simulink model "mpc_psm"  (R2026b)
settings: Solver=ode23tb  StopTime=param.sim.simlength  FixedStep=param.glb_time.tc  MaxStep=param.glb_time.tc
values from neighbouring files (symbols this model uses):
  param = struct()    [init_model.m]
undefined symbols (not defined in the file or in its folder): tc
libraries: fl_lib x28, nesl_utility x13, cstblocks_lti x6, lithium_ion_battery x1, dclink_with_center_tap x1, ideal_bridges_lib x1, dead_time_generator_cmos_simulink x1, single_phase_pwm_modulator x1, threephase_inductor_lib x1, simple_flexible_shaft x1, permanent_magnet_synchronous_machine x1
(part 1 of 3)
settings Model: SimulationMode=accelerator  Creator=dbagn  LastModifiedBy=d.bagnara
settings SolverCC: SolverResetMethod=Robust  ZeroCrossControl=DisableAll
settings DataIOCC: DSMLogging=off  ReturnWorkspaceOutputs=off  SaveOutput=off  SaveTime=off  SignalLogging=off
settings OptimizationCC: ReuseModelBlockBuffer=off
settings SFSimCC: CustomCodeUndefinedFunction=ThrowError  DefaultCustomCodeDeterministicFunctions=All
settings SFSimCC: SimCustomHeaderCode=|
  | #include "rpi.h"
  | #include "mavgflt.h"
  | #include "mavgflt_simulink.h"
  | #include "mavgflts.h"
  | #include "mavgflts_simulink.h"
  | #include "dsmavgflt.h"
  | #include "dsmavgflt_simulink.h"
  | #include "bemf_obsv.h"
  | #include "bemf_obsv_simulink.h"
  | #include "bemf_obsv_load_est.h"
  | #include "bemf_obsv_load_est_simulink.h"
  | #include "dqvector_pi.h"
  | #include "dqvector_pi_simulink.h"
  | #include "sv_pwm_simulink.h"
  | #include "sv_pwm.h"
  | #include "first_harmonic_tracker.h"
  | #include "first_harmonic_tracker_simulink.h"
  | #include "dqpll_thyr.h"
  | #include "dqpll_thyr_simulink.h"
  | #include "dqpll_grid.h"
  | #include "dqpll_grid_simulink.h"
settings SFSimCC: SimUserIncludeDirs=|
  | include
  | src
settings SFSimCC: SimUserSources=|
  | "rpi.c"
  | "mavgflt_simulink.c"
  | "mavgflt.c"
  | "mavgflts_simulink.c"
  | "mavgflts.c"
  | "dsmavgflt_simulink.c"
  | "dsmavgflt.c"
  | "bemf_obsv_simulink.c"
  | "bemf_obsv.c"
  | "bemf_obsv_load_est_simulink.c"
  | "bemf_obsv_load_est.c"
  | "dqvector_pi.c"
  | "dqvector_pi_simulink.c"
  | "sv_pwm_simulink.c"
  | "sv_pwm.c"
  | "first_harmonic_tracker_simulink.c"
  | "first_harmonic_tracker.c"
  | "dqpll_thyr_simulink.c"
  | "dqpll_thyr.c"
  | "dqpll_grid_simulink.c"
  | "dqpll_grid.c"
settings RTWCC: DLArmComputeVersion=19.05
settings SimscapeCC: SimscapeUseEnergyAccounting=off

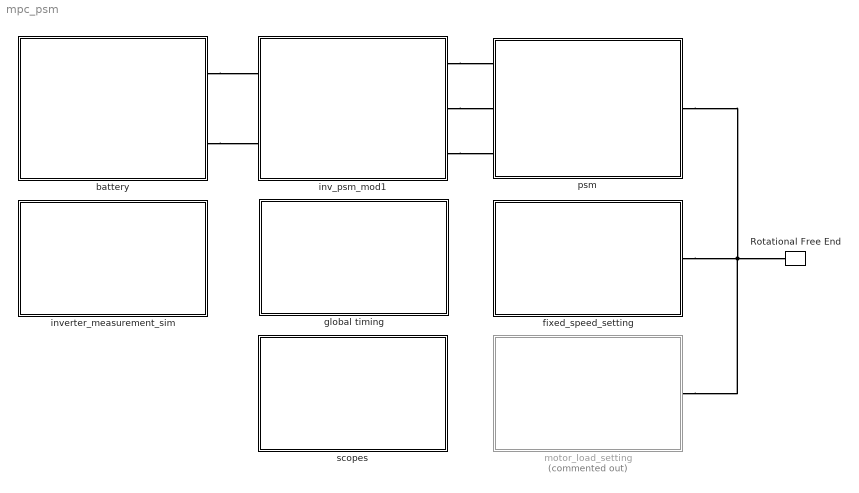
== system mpc_psm ==
  Rotational Free End : fl_lib/Mechanical/Rotational Elements/Rotational Free End  w_specify=off  w_priority=None  w=0 rad/s  w_nominal_specify=off  w_nominal_value=1  w_nominal_unit=rad/s
  battery : Subsystem
  fixed_speed_setting : Subsystem
  global timing : Subsystem
  inv_psm_mod1 : Subsystem
  inverter_measurement_sim : Subsystem
  motor_load_setting : Subsystem  Commented=on
  psm : Subsystem
  scopes : Subsystem
  connections:
  psm/RConn1 -- motor_load_setting/LConn1 -- Rotational Free End/LConn1 -- fixed_speed_setting/LConn1
  inv_psm_mod1/RConn2 -- psm/LConn2
  inv_psm_mod1/RConn1 -- psm/LConn1
  inv_psm_mod1/RConn3 -- psm/LConn3
  battery/RConn1 -- inv_psm_mod1/LConn1
  battery/RConn2 -- inv_psm_mod1/LConn2

== system mpc_psm/battery ==
  Electrical Reference1 : fl_lib/Electrical/Electrical Elements/Electrical Reference
  Solver Configuration : nesl_utility/Solver Configuration  PhysicalDomain=network_engine_domain  SubClassName=solver  LeftPortType=input  RightPortType=generic  Tones=[]  Harmonics=[]  SimulateNoise=off  Profile=off  UseLocalSampling=off  EnableSwitchedLinearOptims=on  FrequencyDomain=off  UseCCode=off  RelTol=0.001  AbsTol=0.001  MinStep=1e-09  ToWorkspace=off  RevertToSquareIcSolve=off  NumHomotopyIterations=100  PhasorMode=off  PhasorModeNumHarmonics=1  ConsistencySolver=NEWTON_FTOL  CanonicalOrdering=UNORDERED  OptimizeIntermediates=UNOPTIMIZED  MulticoreSolverChoice=BACKWARD_EULER  IndexReductionMethod=DerivativeReplacement  DoDC=on  ResidualTolerance=1e-09  ConsistencyTolSource=GLOBAL  ConsistencyAbsTol=0.001  ConsistencyRelTol=0.001  ConsistencyTolFactor=0.001  UseLocalSolver=on  LocalSolverChoice=NE_BACKWARD_EULER_ADVANCER  ResolveIndetEquations=on  FunctionEvalNumThread=1  LocalSolverSampleTime=param.glb_time.tc  DoFixedCost=on  MaxNonlinIter=param.sim.nonlinear_iterations  MaxModeIter=2  ComputeImpulses=off  ImpulseIterations=2  LinearAlgebra=auto  LinearAlgebraNumThread=0  EquationFormulation=NE_TIME_EF  DelaysMemoryBudget=1024  AutomaticFiltering=on  FilteringTimeConstant=0.001  PartitionStorageMethod=AS_NEEDED  PartitionMemoryBudget=1024  PartitionMethod=BALANCED  MultibodyUseLocalSolver=off  MultibodyLocalSolverChoice=ODE1  MultibodyLocalSolverSampleTime=0.001
  To Workspace14 : ToWorkspace  VariableName=battery_data  SampleTime=param.glb_time.tc
      settings: MaxDataPoints=param.glb_time.Nc
  lithium_ion_battery : lithium_ion_battery/lithium_ion_battery  Q=param.battery.pack_1.Q  number_of_cells=param.battery.pack_1.number_of_cells  E_1=param.battery.pack_1.E_1  E0=param.battery.pack_1.E0  E1=param.battery.pack_1.E1  E2=param.battery.pack_1.E2  E3=param.battery.pack_1.E3  Elog=param.battery.pack_1.Elog  R0=param.battery.pack_1.R0  R1=param.battery.pack_1.R1  C1=param.battery.pack_1.C1  M=param.battery.pack_1.M  alpha=param.battery.pack_1.alpha  soc_init=param.battery.pack_1.soc_init  ts_battery=param.glb_time.ts_dab  q1Kalman=param.battery.pack_1.q1Kalman  q2Kalman=param.battery.pack_1.q2Kalman  q3Kalman=param.battery.pack_1.q3Kalman  rKalman=param.battery.pack_1.rKalman  tc=param.glb_time.tc  enable_white_noise_m=0  battery_voltage_init_m=param.battery.nominal_battery_voltage_1
  litium ion battery : Scope
      settings: ActiveDisplayYMinimum=0.16411445056794544  ActiveDisplayYMaximum=0.58434521184828458  DataLoggingVariableName=ScopeData3
  single_phase_ui_measure : Subsystem
  dc+ : PMIOPort  Side=Right
  dc- : PMIOPort  Port=2  Side=Right
  wires:
  lithium_ion_battery/1 -> To Workspace14/1, litium ion battery/1
  connections:
  single_phase_ui_measure/LConn2 -- lithium_ion_battery/RConn2 -- Electrical Reference1/LConn1 -- Solver Configuration/RConn1
  single_phase_ui_measure/RConn1 -- dc+/RConn1
  lithium_ion_battery/RConn1 -- single_phase_ui_measure/LConn1
  dc-/RConn1 -- single_phase_ui_measure/RConn2

== system mpc_psm/fixed_speed_setting ==
  Ideal Angular Velocity Source : fl_lib/Mechanical/Mechanical Sources/Ideal Angular Velocity Source
  Mechanical Rotational Reference : fl_lib/Mechanical/Rotational Elements/Mechanical Rotational Reference
  PS Step1 : fl_lib/Physical Signals/Sources/PS Step  step_time=0.025 s  initial_value=0 rpm  final_value=param.load.rpm_sim rpm
  PS Transfer Function : fl_lib/Physical Signals/Linear Operators/PS Transfer Function  transfer_function_type=foundation.enum.transfer_function_type.lag  T=0.1 s  T1=2 s  T2=1 s  reset_method=foundation.enum.IntegratorResetSpec.None  initial_condition_spec=foundation.enum.IntegratorICSpec.Internal  y0=0 rpm
  shaft : PMIOPort  Side=Left
  connections:
  Mechanical Rotational Reference/LConn1 -- Ideal Angular Velocity Source/RConn2
  PS Step1/RConn1 -- PS Transfer Function/LConn1
  PS Transfer Function/RConn1 -- Ideal Angular Velocity Source/RConn1
  Ideal Angular Velocity Source/LConn1 -- shaft/RConn1

== system mpc_psm/global timing ==
  From9 : From  Commented=on  GotoTag=local_time_corr_afe1
  Unit Delay : UnitDelay  SampleTime=param.glb_time.tc
  Unit Delay1 : UnitDelay  SampleTime=param.glb_time.tc
  time_afe1 : Subsystem  mask{k=param.afe.behav.time_gain_module_1}
      mask prompts: k "Time Gain"
      mask Display:
      | disp('time-gen');
      | port_label('input', 1, 'crt');
      | port_label('output', 1, 'tout');
  time_afe3 : Subsystem  mask{k=1}
      mask prompts: k "Time Gain"
      mask Display:
      | disp('time-gen');
      | port_label('output', 1, 'tout');
  time_inv1 : Subsystem  mask{k=param.inv.behav.time_gain_module_2}
      mask prompts: k "Time Gain"
      mask Display:
      | disp('time-gen');
      | port_label('input', 1, 'crt');
      | port_label('output', 1, 'tout');
  tag scope: time_afe_module_1=global, time_inv_module_1=global, time_master=global
  wires:
  time_afe1/1(Out1) -> [time_afe_module_1]
  time_inv1/1(Out1) -> [time_inv_module_1]
  time_afe3/1(Out1) -> [time_master]
  From9/1 -> Unit Delay/1
  Unit Delay/1 -> time_afe1/1(correction_time)
  [local_time_corr_inv1] -> Unit Delay1/1
  Unit Delay1/1 -> time_inv1/1(correction_time)

== system mpc_psm/inv_psm_mod1 ==
  dclink : Subsystem
  inverter : Subsystem
  inverter_ctrl : Subsystem
  inverter_output_filter : Subsystem
  us_u : PMIOPort  Side=Right
  us_v : PMIOPort  Port=2  Side=Right
  us_w : PMIOPort  Port=3  Side=Right
  udc(+) : PMIOPort  Port=4  Side=Left
  udc(-) : PMIOPort  Port=5  Side=Left
  wires:
  inverter_ctrl/1(cmd_gates) -> inverter/1(cmd_gates)
  connections:
  inverter/LConn2 -- inverter_output_filter/RConn2
  inverter/LConn1 -- inverter_output_filter/RConn1
  inverter/LConn3 -- inverter_output_filter/RConn3
  inverter_output_filter/LConn2 -- us_v/RConn1
  inverter_output_filter/LConn3 -- us_w/RConn1
  inverter_output_filter/LConn1 -- us_u/RConn1
  dclink/RConn1 -- inverter/RConn1
  inverter/RConn2 -- dclink/RConn2
  udc(+)/RConn1 -- dclink/LConn1
  udc(-)/RConn1 -- dclink/LConn2

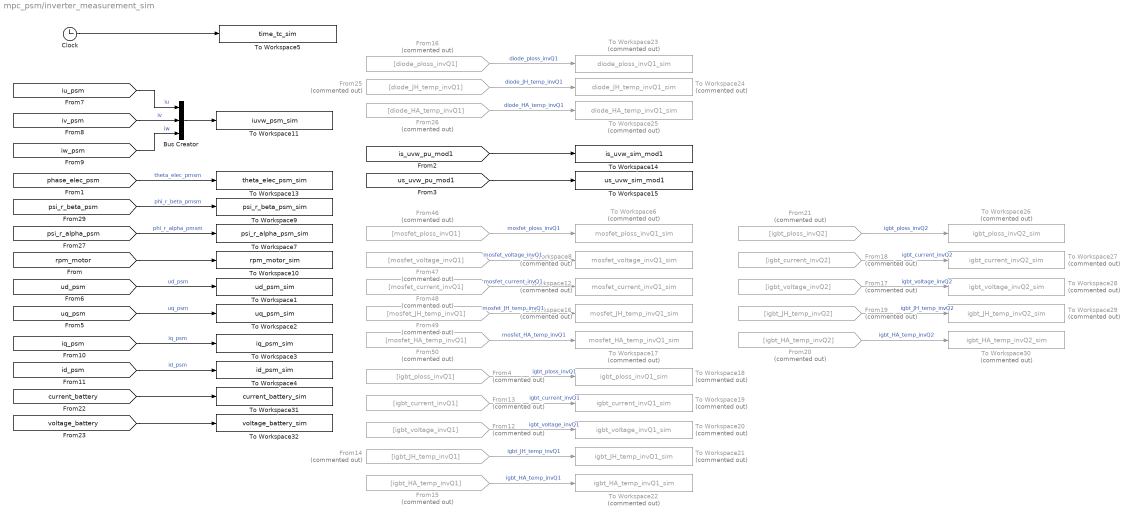
== system mpc_psm/inverter_measurement_sim ==
  Bus Creator : BusCreator  Inputs=3
  Clock : Clock
  From12 : From  Commented=on  GotoTag=igbt_voltage_invQ1
  From13 : From  Commented=on  GotoTag=igbt_current_invQ1
  From14 : From  Commented=on  GotoTag=igbt_JH_temp_invQ1
  From15 : From  Commented=on  GotoTag=igbt_HA_temp_invQ1
  From16 : From  Commented=on  GotoTag=diode_ploss_invQ1
  From17 : From  Commented=on  GotoTag=igbt_voltage_invQ2
  From18 : From  Commented=on  GotoTag=igbt_current_invQ2
  From19 : From  Commented=on  GotoTag=igbt_JH_temp_invQ2
  From20 : From  Commented=on  GotoTag=igbt_HA_temp_invQ2
  From21 : From  Commented=on  GotoTag=igbt_ploss_invQ2
  From25 : From  Commented=on  GotoTag=diode_JH_temp_invQ1
  From26 : From  Commented=on  GotoTag=diode_HA_temp_invQ1
  From4 : From  Commented=on  GotoTag=igbt_ploss_invQ1
  From46 : From  Commented=on  GotoTag=mosfet_ploss_invQ1
  From47 : From  Commented=on  GotoTag=mosfet_voltage_invQ1
  From48 : From  Commented=on  GotoTag=mosfet_current_invQ1
  From49 : From  Commented=on  GotoTag=mosfet_JH_temp_invQ1
  From50 : From  Commented=on  GotoTag=mosfet_HA_temp_invQ1
  To Workspace1 : ToWorkspace  VariableName=ud_psm_sim  SampleTime=param.glb_time.tc
      settings: MaxDataPoints=param.glb_time.Nc  Save2DSignal=2-D array (concatenate along first dimension)
  To Workspace10 : ToWorkspace  VariableName=rpm_motor_sim  SampleTime=param.glb_time.tc
      settings: MaxDataPoints=param.glb_time.Nc  Save2DSignal=2-D array (concatenate along first dimension)
  To Workspace11 : ToWorkspace  VariableName=iuvw_psm_sim  SampleTime=param.glb_time.tc
      settings: MaxDataPoints=param.glb_time.Nc  Save2DSignal=2-D array (concatenate along first dimension)
  To Workspace12 : ToWorkspace  Commented=on  VariableName=mosfet_current_invQ1_sim  SampleTime=tc
      settings: MaxDataPoints=Nc  Save2DSignal=2-D array (concatenate along first dimension)
  To Workspace13 : ToWorkspace  VariableName=theta_elec_psm_sim  SampleTime=param.glb_time.tc
      settings: MaxDataPoints=param.glb_time.Nc  Save2DSignal=2-D array (concatenate along first dimension)
  To Workspace14 : ToWorkspace  VariableName=is_uvw_sim_mod1  SampleTime=param.glb_time.tc
      settings: MaxDataPoints=param.glb_time.Nc  Save2DSignal=2-D array (concatenate along first dimension)
  To Workspace15 : ToWorkspace  VariableName=us_uvw_sim_mod1  SampleTime=param.glb_time.tc
      settings: MaxDataPoints=param.glb_time.Nc  Save2DSignal=2-D array (concatenate along first dimension)
  To Workspace16 : ToWorkspace  Commented=on  VariableName=mosfet_JH_temp_invQ1_sim  SampleTime=tc
      settings: MaxDataPoints=Nc  Save2DSignal=2-D array (concatenate along first dimension)
  To Workspace17 : ToWorkspace  Commented=on  VariableName=mosfet_HA_temp_invQ1_sim  SampleTime=tc
      settings: MaxDataPoints=Nc  Save2DSignal=2-D array (concatenate along first dimension)
  To Workspace18 : ToWorkspace  Commented=on  VariableName=igbt_ploss_invQ1_sim  SampleTime=param.glb_time.tc
      settings: MaxDataPoints=param.glb_time.Nc  Save2DSignal=2-D array (concatenate along first dimension)
  To Workspace19 : ToWorkspace  Commented=on  VariableName=igbt_current_invQ1_sim  SampleTime=param.glb_time.tc
      settings: MaxDataPoints=param.glb_time.Nc  Save2DSignal=2-D array (concatenate along first dimension)
  To Workspace2 : ToWorkspace  VariableName=uq_psm_sim  SampleTime=param.glb_time.tc
      settings: MaxDataPoints=param.glb_time.Nc  Save2DSignal=2-D array (concatenate along first dimension)
  To Workspace20 : ToWorkspace  Commented=on  VariableName=igbt_voltage_invQ1_sim  SampleTime=param.glb_time.tc
      settings: MaxDataPoints=param.glb_time.Nc  Save2DSignal=2-D array (concatenate along first dimension)
  To Workspace21 : ToWorkspace  Commented=on  VariableName=igbt_JH_temp_invQ1_sim  SampleTime=param.glb_time.tc
      settings: MaxDataPoints=param.glb_time.Nc  Save2DSignal=2-D array (concatenate along first dimension)
  To Workspace22 : ToWorkspace  Commented=on  VariableName=igbt_HA_temp_invQ1_sim  SampleTime=param.glb_time.tc
      settings: MaxDataPoints=param.glb_time.Nc  Save2DSignal=2-D array (concatenate along first dimension)
  To Workspace23 : ToWorkspace  Commented=on  VariableName=diode_ploss_invQ1_sim  SampleTime=param.glb_time.tc
      settings: MaxDataPoints=param.glb_time.Nc
  To Workspace24 : ToWorkspace  Commented=on  VariableName=diode_JH_temp_invQ1_sim  SampleTime=param.glb_time.tc
      settings: MaxDataPoints=param.glb_time.Nc
  To Workspace25 : ToWorkspace  Commented=on  VariableName=diode_HA_temp_invQ1_sim  SampleTime=param.glb_time.tc
      settings: MaxDataPoints=param.glb_time.Nc
  To Workspace26 : ToWorkspace  Commented=on  VariableName=igbt_ploss_invQ2_sim  SampleTime=param.glb_time.tc
      settings: MaxDataPoints=param.glb_time.Nc  Save2DSignal=2-D array (concatenate along first dimension)
  To Workspace27 : ToWorkspace  Commented=on  VariableName=igbt_current_invQ2_sim  SampleTime=param.glb_time.tc
      settings: MaxDataPoints=param.glb_time.Nc  Save2DSignal=2-D array (concatenate along first dimension)
  To Workspace28 : ToWorkspace  Commented=on  VariableName=igbt_voltage_invQ2_sim  SampleTime=param.glb_time.tc
      settings: MaxDataPoints=param.glb_time.Nc  Save2DSignal=2-D array (concatenate along first dimension)
  To Workspace29 : ToWorkspace  Commented=on  VariableName=igbt_JH_temp_invQ2_sim  SampleTime=param.glb_time.tc
      settings: MaxDataPoints=param.glb_time.Nc  Save2DSignal=2-D array (concatenate along first dimension)
  To Workspace3 : ToWorkspace  VariableName=iq_psm_sim  SampleTime=param.glb_time.tc
      settings: MaxDataPoints=param.glb_time.Nc  Save2DSignal=2-D array (concatenate along first dimension)
  To Workspace30 : ToWorkspace  Commented=on  VariableName=igbt_HA_temp_invQ2_sim  SampleTime=param.glb_time.tc
      settings: MaxDataPoints=param.glb_time.Nc  Save2DSignal=2-D array (concatenate along first dimension)
  To Workspace31 : ToWorkspace  VariableName=current_battery_sim  SampleTime=param.glb_time.tc
      settings: MaxDataPoints=param.glb_time.Nc  Save2DSignal=2-D array (concatenate along first dimension)
  To Workspace32 : ToWorkspace  VariableName=voltage_battery_sim  SampleTime=param.glb_time.tc
      settings: MaxDataPoints=param.glb_time.Nc  Save2DSignal=2-D array (concatenate along first dimension)
  To Workspace4 : ToWorkspace  VariableName=id_psm_sim  SampleTime=param.glb_time.tc
      settings: MaxDataPoints=param.glb_time.Nc  Save2DSignal=2-D array (concatenate along first dimension)
  To Workspace5 : ToWorkspace  VariableName=time_tc_sim  SampleTime=param.glb_time.tc
      settings: MaxDataPoints=param.glb_time.Nc  Save2DSignal=2-D array (concatenate along first dimension)
  To Workspace6 : ToWorkspace  Commented=on  VariableName=mosfet_ploss_invQ1_sim  SampleTime=tc
      settings: MaxDataPoints=Nc  Save2DSignal=2-D array (concatenate along first dimension)
  To Workspace7 : ToWorkspace  VariableName=psi_r_alpha_psm_sim  SampleTime=param.glb_time.tc
      settings: MaxDataPoints=param.glb_time.Nc  Save2DSignal=2-D array (concatenate along first dimension)
  To Workspace8 : ToWorkspace  Commented=on  VariableName=mosfet_voltage_invQ1_sim  SampleTime=tc
      settings: MaxDataPoints=Nc  Save2DSignal=2-D array (concatenate along first dimension)
  To Workspace9 : ToWorkspace  VariableName=psi_r_beta_psm_sim  SampleTime=param.glb_time.tc
      settings: MaxDataPoints=param.glb_time.Nc  Save2DSignal=2-D array (concatenate along first dimension)
  wires:
  [psi_r_alpha_psm] -> To Workspace7/1  "phi_r_alpha_pmsm"
  [psi_r_beta_psm] -> To Workspace9/1  "phi_r_beta_pmsm"
  [rpm_motor] -> To Workspace10/1
  [iv_psm] -> Bus Creator/2  "iv"
  [iw_psm] -> Bus Creator/3  "iw"
  [iu_psm] -> Bus Creator/1  "iu"
  Bus Creator/1 -> To Workspace11/1
  [phase_elec_psm] -> To Workspace13/1  "theta_elec_pmsm"
  [ud_psm] -> To Workspace1/1  "ud_psm"
  [uq_psm] -> To Workspace2/1  "uq_psm"
  [iq_psm] -> To Workspace3/1  "iq_psm"
  [id_psm] -> To Workspace4/1  "id_psm"
  Clock/1 -> To Workspace5/1
  From46/1 -> To Workspace6/1  "mosfet_ploss_invQ1"
  From49/1 -> To Workspace16/1  "mosfet_JH_temp_invQ1"
  From50/1 -> To Workspace17/1  "mosfet_HA_temp_invQ1"
  [is_uvw_pu_mod1] -> To Workspace14/1
  [us_uvw_pu_mod1] -> To Workspace15/1
  From47/1 -> To Workspace8/1  "mosfet_voltage_invQ1"
  From48/1 -> To Workspace12/1  "mosfet_current_invQ1"
  From4/1 -> To Workspace18/1  "igbt_ploss_invQ1"
  From13/1 -> To Workspace19/1  "igbt_current_invQ1"
  From12/1 -> To Workspace20/1  "igbt_voltage_invQ1"
  From14/1 -> To Workspace21/1  "igbt_JH_temp_invQ1"
  From15/1 -> To Workspace22/1  "igbt_HA_temp_invQ1"
  From16/1 -> To Workspace23/1  "diode_ploss_invQ1"
  From25/1 -> To Workspace24/1  "diode_JH_temp_invQ1"
  From26/1 -> To Workspace25/1  "diode_HA_temp_invQ1"
  From20/1 -> To Workspace30/1  "igbt_HA_temp_invQ2"
  From19/1 -> To Workspace29/1  "igbt_JH_temp_invQ2"
  From17/1 -> To Workspace28/1  "igbt_voltage_invQ2"
  From18/1 -> To Workspace27/1  "igbt_current_invQ2"
  From21/1 -> To Workspace26/1  "igbt_ploss_invQ2"
  [current_battery] -> To Workspace31/1
  [voltage_battery] -> To Workspace32/1

== system mpc_psm/motor_load_setting ==
  Ideal Torque Source : fl_lib/Mechanical/Mechanical Sources/Ideal Torque Source
  Inertia : fl_lib/Mechanical/Rotational Elements/Inertia  inertia=param.load.external_load_inertia kg*m^2  num_ports=foundation.enum.numPorts2.one  w_specify=off  w_priority=High  w=0 rad/s  w_nominal_specify=off  w_nominal_value=1  w_nominal_unit=rad/s  t_specify=off  t_priority=None  t=0 N*m  t_nominal_specify=off  t_nominal_value=1  t_nominal_unit=N*m
  Mechanical Rotational Reference : fl_lib/Mechanical/Rotational Elements/Mechanical Rotational Reference
  PS Step : fl_lib/Physical Signals/Sources/PS Step  step_time=param.sim.load_step_time s  initial_value=1 N*m  final_value=1 N*m
  PS Transfer Function : fl_lib/Physical Signals/Linear Operators/PS Transfer Function  transfer_function_type=foundation.enum.transfer_function_type.lag  T=1 s  T1=2 s  T2=1 s  reset_method=foundation.enum.IntegratorResetSpec.None  initial_condition_spec=foundation.enum.IntegratorICSpec.Internal  y0=0 N*m
  flexible_shaft : simple_flexible_shaft/flexible_shaft  b1=1  b2=1  J1=1  J2=1  b_displacement=1  k_displacement=1e5
  shaft : PMIOPort  Side=Left
  connections:
  Ideal Torque Source/LConn1 -- flexible_shaft/RConn1 -- Inertia/LConn1
  Ideal Torque Source/RConn2 -- Mechanical Rotational Reference/LConn1
  PS Transfer Function/RConn1 -- Ideal Torque Source/RConn1
  PS Step/RConn1 -- PS Transfer Function/LConn1
  flexible_shaft/LConn1 -- shaft/RConn1

== system mpc_psm/psm ==
  Bus Selector1 : BusSelector  OutputSignals=omega_mech (rpm)
  Constant : Constant  Value=param.psm.machine.psi_m
  Simulink-PS Converter3 : nesl_utility/Simulink-PS Converter  PhysicalDomain=network_engine_domain  SubClassName=ps_input  LeftPortType=input  RightPortType=output  PseudoPeriodic=off  Frequencies=[]  NoiseDistribution=none  NoiseParameters=[]  Unit=V*s  AffineConversion=on  FilteringAndDerivatives=provide  SimscapeFilterOrder=1  InputFilterTimeConstant=0.001  UdotUserProvided=0
  synchronous_motor : Subsystem
  u : PMIOPort  Side=Left
  v : PMIOPort  Port=2  Side=Left
  w : PMIOPort  Port=3  Side=Left
  shaft : PMIOPort  Port=4  Side=Right
  tag scope: rpm_motor=global
  wires:
  synchronous_motor/1(motor_data) -> Bus Selector1/1
  Bus Selector1/1 -> [rpm_motor]  "<omega_mech (rpm)>"
  Constant/1 -> Simulink-PS Converter3/1
  connections:
  synchronous_motor/LConn1 -- u/RConn1
  Simulink-PS Converter3/RConn1 -- synchronous_motor/LConn4
  synchronous_motor/LConn3 -- w/RConn1
  synchronous_motor/LConn2 -- v/RConn1
  shaft/RConn1 -- synchronous_motor/RConn1

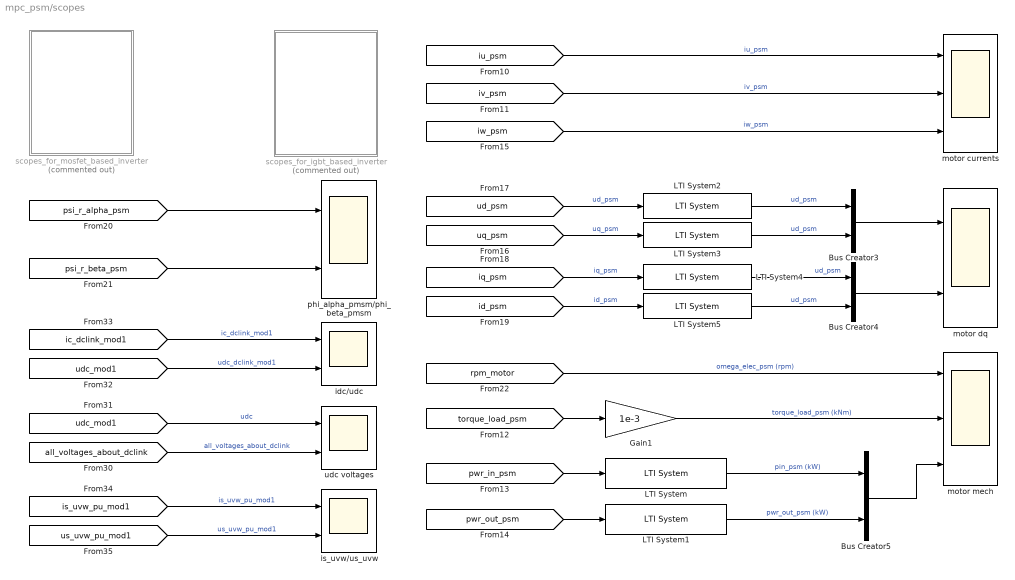
== system mpc_psm/scopes ==
  Bus Creator3 : BusCreator  Inputs=2
  Bus Creator4 : BusCreator  Inputs=2
  Bus Creator5 : BusCreator  Inputs=2
  Gain1 : Gain  Gain=1e-3
  LTI System{,1..5} (6 alike) : cstblocks_lti/LTI System  sys=param.ctrl.filters.inv.SOF_50Hz.ss_c  IC=[]  PadeOrder=0
  idc/udc : Scope  NumInputPorts=2
      settings: SampleTime=param.glb_time.tc  ActiveDisplayYMinimum=-429.79232670429462  ActiveDisplayYMaximum=486.89839586541632  DataLoggingVariableName=ScopeData23
  is_uvw/us_uvw : Scope  NumInputPorts=2
      settings: SampleTime=param.glb_time.tc  ActiveDisplayYMinimum=-4.0901889520524559  ActiveDisplayYMaximum=4.1379165768312332  DataLoggingVariableName=ScopeData25
  motor currents : Scope  NumInputPorts=3
      settings: SampleTime=param.glb_time.tc  ActiveDisplayYMinimum=58.424845691421581  ActiveDisplayYMaximum=93.288598080369269  DataLoggingVariableName=ScopeData17
  motor dq : Scope  NumInputPorts=2
      settings: SampleTime=param.glb_time.tc  ActiveDisplayYMinimum=-581.89506711994022  ActiveDisplayYMaximum=671.86127351087941  DataLoggingVariableName=ScopeData18
  motor mech : Scope  NumInputPorts=3
      settings: SampleTime=param.glb_time.tc  ActiveDisplayYMinimum=17.183598515360881  ActiveDisplayYMaximum=17.193981269957806  DataLoggingVariableName=ScopeData11
  phi_alpha_pmsm/phi_beta_pmsm : Scope  NumInputPorts=2
      settings: SampleTime=param.glb_time.tc  ActiveDisplayYMinimum=-4.800821748013445  ActiveDisplayYMaximum=4.8008423854253959  DataLoggingVariableName=ScopeData19
  scopes_for_igbt_based_inverter : Subsystem  Commented=on
  scopes_for_mosfet_based_inverter : Subsystem  Commented=on
  udc voltages : Scope  NumInputPorts=2
      settings: SampleTime=param.glb_time.tc  ActiveDisplayYMinimum=1171.2930142420437  ActiveDisplayYMaximum=1182.3226675773467  DataLoggingVariableName=ScopeData24
  wires:
  [torque_load_psm] -> Gain1/1
  [pwr_out_psm] -> LTI System1/1
  Bus Creator4/1 -> motor dq/2
  LTI System/1 -> Bus Creator5/1  "pin_psm (kW)"
  LTI System1/1 -> Bus Creator5/2  "pwr_out_psm (kW)"
  [iw_psm] -> motor currents/3  "iw_psm"
  Gain1/1 -> motor mech/2  "torque_load_psm (kNm)"
  [id_psm] -> LTI System5/1  "id_psm"
  [psi_r_alpha_psm] -> phi_alpha_pmsm/phi_beta_pmsm/1
  [iv_psm] -> motor currents/2  "iv_psm"
  Bus Creator3/1 -> motor dq/1
  [uq_psm] -> LTI System3/1  "uq_psm"
  [iu_psm] -> motor currents/1  "iu_psm"
  Bus Creator5/1 -> motor mech/3
  [ud_psm] -> LTI System2/1  "ud_psm"
  [iq_psm] -> LTI System4/1  "iq_psm"
  [rpm_motor] -> motor mech/1  "omega_elec_psm (rpm)"
  [pwr_in_psm] -> LTI System/1
  [psi_r_beta_psm] -> phi_alpha_pmsm/phi_beta_pmsm/2
  [udc_mod1] -> udc voltages/1  "udc"
  [ic_dclink_mod1] -> idc/udc/1  "ic_dclink_mod1"
  [udc_mod1] -> idc/udc/2  "udc_dclink_mod1"
  [all_voltages_about_dclink] -> udc voltages/2  "all_voltages_about_dclink"
  [is_uvw_pu_mod1] -> is_uvw/us_uvw/1  "is_uvw_pu_mod1"
  [us_uvw_pu_mod1] -> is_uvw/us_uvw/2  "us_uvw_pu_mod1"
  LTI System2/1 -> Bus Creator3/1  "ud_psm"
  LTI System3/1 -> Bus Creator3/2  "ud_psm"
  LTI System4/1 -> Bus Creator4/1  "ud_psm"
  LTI System5/1 -> Bus Creator4/2  "ud_psm"

== system mpc_psm/battery/single_phase_ui_measure ==
  Bus Creator : BusCreator  Inputs=2
  Current Sensor : fl_lib/Electrical/Electrical Sensors/Current Sensor
  Selector : Selector  InputPortWidth=2  IndexOptions=Index vector (dialog)  Indices=2  OutputSizes=1  RuntimeRangeChecks=off
  Selector1 : Selector  InputPortWidth=2  IndexOptions=Index vector (dialog)  Indices=1  OutputSizes=1  RuntimeRangeChecks=off
  Voltage Sensor : fl_lib/Electrical/Electrical Sensors/Voltage Sensor
  dab input modA : Scope  NumInputPorts=2
      settings: SampleTime=param.glb_time.tc  ActiveDisplayYMinimum=-0.63173529794617089  ActiveDisplayYMaximum=0.79076436133006256  DataLoggingVariableName=ScopeData2
  iph : nesl_utility/PS-Simulink Converter  PhysicalDomain=network_engine_domain  SubClassName=ps_output  LeftPortType=input  RightPortType=output  PseudoPeriodic=off  Frequencies=[]  VectorFormat=1-D array  Unit=A  AffineConversion=off
  uph : nesl_utility/PS-Simulink Converter  PhysicalDomain=network_engine_domain  SubClassName=ps_output  LeftPortType=input  RightPortType=output  PseudoPeriodic=off  Frequencies=[]  VectorFormat=1-D array  Unit=V  AffineConversion=off
  Udc(+) : PMIOPort  Side=Left
  udc(+) : PMIOPort  Port=2  Side=Right
  Udc(-) : PMIOPort  Port=3  Side=Left
  udc(-) : PMIOPort  Port=4  Side=Right
  tag scope: current_battery=global, voltage_battery=global
  wires:
  Bus Creator/1 -> Selector/1, Selector1/1  "ui_data"
  iph/1 -> Bus Creator/1  "iph"
  uph/1 -> Bus Creator/2  "uph"
  Selector1/1 -> [current_battery], dab input modA/1  "current_battery"
  Selector/1 -> dab input modA/2, [voltage_battery]  "voltage_battery"
  connections:
  iph/LConn1 -- Current Sensor/RConn1
  Voltage Sensor/LConn1 -- Current Sensor/LConn1 -- Udc(+)/RConn1
  Current Sensor/RConn2 -- udc(+)/RConn1
  Voltage Sensor/RConn1 -- uph/LConn1
  Voltage Sensor/RConn2 -- Udc(-)/RConn1 -- udc(-)/RConn1

== system mpc_psm/global timing/time_afe1 ==
  correction_time : Inport
  Constant : Constant
  Gain : Gain  Gain=k
  Product : Product
  Sum : Sum  Inputs=|++
  time_1 : Clock
  Out1 : Outport
  wires:
  time_1/1 -> Gain/1
  Gain/1 -> Product/1
  Product/1 -> Out1/1
  correction_time/1 -> Sum/1
  Sum/1 -> Product/2
  Constant/1 -> Sum/2

== system mpc_psm/global timing/time_afe3 ==
  Gain : Gain  Gain=k
  time_1 : Clock
  Out1 : Outport
  wires:
  Gain/1 -> Out1/1
  time_1/1 -> Gain/1

== system mpc_psm/global timing/time_inv1 ==
  correction_time : Inport
  Constant : Constant
  Gain : Gain  Gain=k
  Product : Product
  Sum : Sum  Inputs=|++
  time_1 : Clock
  Out1 : Outport
  wires:
  time_1/1 -> Gain/1
  Gain/1 -> Product/1
  Product/1 -> Out1/1
  correction_time/1 -> Sum/1
  Constant/1 -> Sum/2
  Sum/1 -> Product/2

== system mpc_psm/inv_psm_mod1/dclink ==
  Bus Selector : BusSelector  OutputSignals=udc,Cdc1_current,vdc_pu
  Electrical Reference : fl_lib/Electrical/Electrical Elements/Electrical Reference
  dclink : dclink_with_center_tap/dclink  Cdc1=param.inv.hw.CFi1  Cdc2=param.inv.hw.CFi2  Rudc_measure=107e3  Vdc_scale=param.inv.hw.udc_nom
  udc(+) : PMIOPort  Side=Right
  udc(-) : PMIOPort  Port=2  Side=Right
  Udc(+) : PMIOPort  Port=3  Side=Left
  Udc(-) : PMIOPort  Port=4  Side=Left
  tag scope: all_voltages_about_dclink=global, ic_dclink_mod1=global, udc_mod1=global, vdc_pu_inv_mod1=global
  wires:
  dclink/1 -> Bus Selector/1, [all_voltages_about_dclink]
  Bus Selector/1 -> [udc_mod1]  "<udc>"
  Bus Selector/2 -> [ic_dclink_mod1]  "<Cdc1_current>"
  Bus Selector/3 -> [vdc_pu_inv_mod1]  "<vdc_pu>"
  connections:
  dclink/LConn1 -- udc(+)/RConn1
  Electrical Reference/LConn1 -- dclink/RConn2
  udc(-)/RConn1 -- dclink/LConn2
  Udc(+)/RConn1 -- dclink/RConn1
  Udc(-)/RConn1 -- dclink/RConn3

== system mpc_psm/inv_psm_mod1/inverter ==
  cmd_gates : Inport
  Current Sensor : fl_lib/Electrical/Electrical Sensors/Current Sensor
  PS-Simulink Converter1 : nesl_utility/PS-Simulink Converter  PhysicalDomain=network_engine_domain  SubClassName=ps_output  LeftPortType=input  RightPortType=output  PseudoPeriodic=off  Frequencies=[]  VectorFormat=1-D array  Unit=A  AffineConversion=on
  PS-Simulink Converter4 : nesl_utility/PS-Simulink Converter  PhysicalDomain=network_engine_domain  SubClassName=ps_output  LeftPortType=input  RightPortType=output  PseudoPeriodic=off  Frequencies=[]  VectorFormat=1-D array  Unit=V  AffineConversion=on
  To Workspace : ToWorkspace  VariableName=idc_sim_mod1  SampleTime=param.glb_time.tc
      settings: MaxDataPoints=param.glb_time.Nc
  To Workspace1 : ToWorkspace  VariableName=udc_sim_mod1  SampleTime=param.glb_time.tc
      settings: MaxDataPoints=param.glb_time.Nc
  Transfer Fcn : TransferFcn  Denominator=[1e-2 1]
  Voltage Sensor : fl_lib/Electrical/Electrical Sensors/Voltage Sensor
  idc/udc : Scope  NumInputPorts=2
      settings: SampleTime=param.glb_time.tc  ActiveDisplayYMinimum=-35.22322330009689  ActiveDisplayYMaximum=317.00900970087207
  inverter : Subsystem
  Udc(+) : PMIOPort  Side=Right
  Udc(-) : PMIOPort  Port=2  Side=Right
  us_u : PMIOPort  Port=3  Side=Left
  us_v : PMIOPort  Port=4  Side=Left
  us_w : PMIOPort  Port=5  Side=Left
  wires:
  PS-Simulink Converter4/1 -> To Workspace1/1, idc/udc/2  "udc"
  PS-Simulink Converter1/1 -> Transfer Fcn/1  "idc"
  Transfer Fcn/1 -> To Workspace/1, idc/udc/1  "idc_flt"
  cmd_gates/1 -> inverter/1(gate_cmds_uvw)
  connections:
  PS-Simulink Converter4/LConn1 -- Voltage Sensor/RConn1
  us_u/RConn1 -- inverter/LConn1
  us_v/RConn1 -- inverter/LConn2
  us_w/RConn1 -- inverter/LConn3
  Voltage Sensor/RConn2 -- Udc(-)/RConn1 -- inverter/RConn2
  Current Sensor/LConn1 -- Udc(+)/RConn1
  Voltage Sensor/LConn1 -- inverter/RConn1 -- Current Sensor/RConn2
  PS-Simulink Converter1/LConn1 -- Current Sensor/RConn1

== system mpc_psm/inv_psm_mod1/inverter_ctrl ==
  inverter_control : Subsystem
  cmd_gates : Outport
  tag scope: local_time_corr_inv1=global, master_torque_ref=global
  wires:
  [is_uvw_pu_mod1] -> inverter_control/1(is_uvw)
  [TRGO_inv_module_1] -> inverter_control/Trigger
  [vdc_pu_inv_mod1] -> inverter_control/2(udc_pu)
  inverter_control/1(cmd_gates) -> cmd_gates/1
  [time_inv_module_1] -> inverter_control/3(local_time)
  [time_master] -> inverter_control/4(master_time)
  inverter_control/2(local_time_corr) -> [local_time_corr_inv1]
  inverter_control/3(master_torque_ref) -> [master_torque_ref]
  [phase_elec_psm] -> inverter_control/5(theta_elec_psm)
  [omega_elec_psm] -> inverter_control/6(omega_elec_psm)

== system mpc_psm/inv_psm_mod1/inverter_output_filter ==
  Inductor : fl_lib/Electrical/Electrical Elements/Inductor  l=1e-6 H  r=0 Ohm  g=1e-9 1/Ohm  i_specify=off  i_priority=None  i=0 A  i_nominal_specify=off  i_nominal_value=1  i_nominal_unit=A  v_specify=off  v_priority=None  v=0 V  v_nominal_specify=off  v_nominal_value=1  v_nominal_unit=V  i_L_specify=off  i_L_priority=High  i_L=0 A  i_L_nominal_specify=off  i_L_nominal_value=1  i_L_nominal_unit=A
  Inductor1 : fl_lib/Electrical/Electrical Elements/Inductor  l=1e-6 H  r=0 Ohm  g=1e-9 1/Ohm  i_specify=off  i_priority=None  i=0 A  i_nominal_specify=off  i_nominal_value=1  i_nominal_unit=A  v_specify=off  v_priority=None  v=0 V  v_nominal_specify=off  v_nominal_value=1  v_nominal_unit=V  i_L_specify=off  i_L_priority=High  i_L=0 A  i_L_nominal_specify=off  i_L_nominal_value=1  i_L_nominal_unit=A
  Inductor2 : fl_lib/Electrical/Electrical Elements/Inductor  l=1e-6 H  r=0 Ohm  g=1e-9 1/Ohm  i_specify=off  i_priority=None  i=0 A  i_nominal_specify=off  i_nominal_value=1  i_nominal_unit=A  v_specify=off  v_priority=None  v=0 V  v_nominal_specify=off  v_nominal_value=1  v_nominal_unit=V  i_L_specify=off  i_L_priority=High  i_L=0 A  i_L_nominal_specify=off  i_L_nominal_value=1  i_L_nominal_unit=A
  threephase inductor : threephase_inductor_lib/threephase inductor  Lp=param.inv.hw.LFi H  L0=param.inv.hw.LFi_cm H  Rp=param.inv.hw.RLFi Ohm  R0=param.inv.hw.RLFi_cm Ohm  Lls=5e-6 H  uu_1_specify=off  uu_1_priority=None  uu_1=0 V  uu_1_nominal_specify=off  uu_1_nominal_value=1  uu_1_nominal_unit=V  uv_1_specify=off  uv_1_priority=None  uv_1=0 V  uv_1_nominal_specify=off  uv_1_nominal_value=1  uv_1_nominal_unit=V  uw_1_specify=off  uw_1_priority=None  uw_1=0 V  uw_1_nominal_specify=off  uw_1_nominal_value=1  uw_1_nominal_unit=V  uu_2_specify=off  uu_2_priority=None  uu_2=0 V  uu_2_nominal_specify=off  uu_2_nominal_value=1  uu_2_nominal_unit=V  uv_2_specify=off  uv_2_priority=None  uv_2=0 V  uv_2_nominal_specify=off  uv_2_nominal_value=1  uv_2_nominal_unit=V  uw_2_specify=off  uw_2_priority=None  uw_2=0 V  uw_2_nominal_specify=off  uw_2_nominal_value=1  uw_2_nominal_unit=V  iu_specify=off  iu_priority=None  iu=0 A  iu_nominal_specify=off  iu_nominal_value=1  iu_nominal_unit=A  iv_specify=off  iv_priority=None  iv=0 A  iv_nominal_specify=off  iv_nominal_value=1  iv_nominal_unit=A  iw_specify=off  iw_priority=None  iw=0 A  iw_nominal_specify=off  iw_nominal_value=1  iw_nominal_unit=A
  threephase_vi_measures_stack : Subsystem
  us_u : PMIOPort  Side=Left
  uu : PMIOPort  Port=2  Side=Right
  us_v : PMIOPort  Port=3  Side=Left
  uv : PMIOPort  Port=4  Side=Right
  us_w : PMIOPort  Port=5  Side=Left
  uw : PMIOPort  Port=6  Side=Right
  connections:
  threephase_vi_measures_stack/LConn1 -- us_u/RConn1
  threephase_vi_measures_stack/LConn2 -- us_v/RConn1
  threephase_vi_measures_stack/LConn3 -- us_w/RConn1
  threephase inductor/LConn1 -- threephase_vi_measures_stack/RConn1
  threephase inductor/LConn2 -- threephase_vi_measures_stack/RConn2
  threephase inductor/LConn3 -- threephase_vi_measures_stack/RConn3
  threephase inductor/RConn1 -- Inductor/LConn1
  threephase inductor/RConn2 -- Inductor1/LConn1
  threephase inductor/RConn3 -- Inductor2/LConn1
  Inductor/RConn1 -- uu/RConn1
  Inductor1/RConn1 -- uv/RConn1
  Inductor2/RConn1 -- uw/RConn1

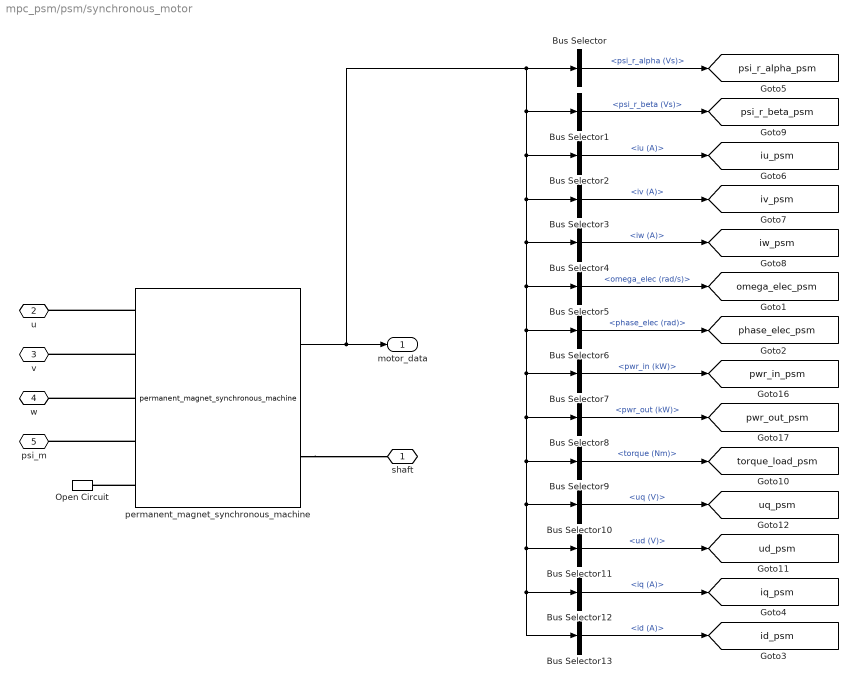
== system mpc_psm/psm/synchronous_motor ==
  Bus Selector : BusSelector  OutputSignals=psi_r_alpha (Vs)
  Bus Selector1 : BusSelector  OutputSignals=psi_r_beta (Vs)
  Bus Selector10 : BusSelector  OutputSignals=uq (V)
  Bus Selector11 : BusSelector  OutputSignals=ud (V)
  Bus Selector12 : BusSelector  OutputSignals=iq (A)
  Bus Selector13 : BusSelector  OutputSignals=id (A)
  Bus Selector2 : BusSelector  OutputSignals=iu (A)
  Bus Selector3 : BusSelector  OutputSignals=iv (A)
  Bus Selector4 : BusSelector  OutputSignals=iw (A)
  Bus Selector5 : BusSelector  OutputSignals=omega_elec (rad/s)
  Bus Selector6 : BusSelector  OutputSignals=phase_elec (rad)
  Bus Selector7 : BusSelector  OutputSignals=pwr_in (kW)
  Bus Selector8 : BusSelector  OutputSignals=pwr_out (kW)
  Bus Selector9 : BusSelector  OutputSignals=torque (Nm)
  Open Circuit : fl_lib/Electrical/Electrical Elements/Open Circuit  v_specify=off  v_priority=None  v=0 V  v_nominal_specify=off  v_nominal_value=1  v_nominal_unit=V
  permanent_magnet_synchronous_machine : permanent_magnet_synchronous_machine/permanent_magnet_synchronous_machine  pp=param.psm.machine.number_poles  psi_m=param.psm.machine.psi_m  Lmu=param.psm.machine.Lmu  La=param.psm.machine.La_m  Lb=param.psm.machine.Lb_m  Rs=param.psm.machine.Rs_m  Jm=param.psm.machine.Jm_m  b_linear=param.psm.machine.load_friction_m  b_quadratic=0  h5_percent=0  h7_percent=0  psi_r_u_init=param.psm.machine.psi_m  psi_r_v_init=-param.psm.machine.psi_m/2  psi_r_w_init=-param.psm.machine.psi_m/2  omega_init=0  phase_init=0  angle_error=0
  shaft : PMIOPort  Side=Right
  u : PMIOPort  Port=2  Side=Left
  v : PMIOPort  Port=3  Side=Left
  w : PMIOPort  Port=4  Side=Left
  psi_m : PMIOPort  Port=5  Side=Left
  motor_data : Outport
  tag scope: id_psm=global, iq_psm=global, iu_psm=global, iv_psm=global, iw_psm=global, omega_elec_psm=global, phase_elec_psm=global, psi_r_alpha_psm=global, psi_r_beta_psm=global, pwr_in_psm=global, pwr_out_psm=global, torque_load_psm=global, ud_psm=global, uq_psm=global
  wires:
  permanent_magnet_synchronous_machine/1 -> Bus Selector8/1, Bus Selector10/1, Bus Selector11/1, Bus Selector12/1, Bus Selector13/1, Bus Selector9/1, Bus Selector7/1, Bus Selector6/1, Bus Selector5/1, Bus Selector4/1, Bus Selector3/1, Bus Selector2/1, Bus Selector1/1, Bus Selector/1, motor_data/1
  Bus Selector/1 -> [psi_r_alpha_psm]  "<psi_r_alpha (Vs)>"
  Bus Selector1/1 -> [psi_r_beta_psm]  "<psi_r_beta (Vs)>"
  Bus Selector2/1 -> [iu_psm]  "<iu (A)>"
  Bus Selector3/1 -> [iv_psm]  "<iv (A)>"
  Bus Selector4/1 -> [iw_psm]  "<iw (A)>"
  Bus Selector5/1 -> [omega_elec_psm]  "<omega_elec (rad/s)>"
  Bus Selector6/1 -> [phase_elec_psm]  "<phase_elec (rad)>"
  Bus Selector7/1 -> [pwr_in_psm]  "<pwr_in (kW)>"
  Bus Selector8/1 -> [pwr_out_psm]  "<pwr_out (kW)>"
  Bus Selector9/1 -> [torque_load_psm]  "<torque (Nm)>"
  Bus Selector10/1 -> [uq_psm]  "<uq (V)>"
  Bus Selector11/1 -> [ud_psm]  "<ud (V)>"
  Bus Selector12/1 -> [iq_psm]  "<iq (A)>"
  Bus Selector13/1 -> [id_psm]  "<id (A)>"
  connections:
  permanent_magnet_synchronous_machine/RConn1 -- shaft/RConn1
  permanent_magnet_synchronous_machine/LConn1 -- u/RConn1
  permanent_magnet_synchronous_machine/LConn2 -- v/RConn1
  permanent_magnet_synchronous_machine/LConn3 -- w/RConn1
  permanent_magnet_synchronous_machine/LConn4 -- psi_m/RConn1
  permanent_magnet_synchronous_machine/LConn5 -- Open Circuit/LConn1

== system mpc_psm/scopes/scopes_for_igbt_based_inverter ==
  Bus Creator1 : BusCreator  Inputs=2
  Bus Creator2 : BusCreator  Inputs=2
  Bus Creator6 : BusCreator  Inputs=2
  diode power losses INV Q1 : Scope  NumInputPorts=2
      settings: SampleTime=param.glb_time.tc  ActiveDisplayYMinimum=-1.5240099779957812  ActiveDisplayYMaximum=13.716019351034738  DataLoggingVariableName=ScopeData4
  igbt power losses INV Q1 : Scope  NumInputPorts=4
      settings: SampleTime=param.glb_time.tc  ActiveDisplayYMinimum=-146.40069949224531  ActiveDisplayYMaximum=1321.3065614948737  DataLoggingVariableName=ScopeData16
  igbt power losses INV Q2 : Scope  NumInputPorts=4
      settings: SampleTime=param.glb_time.tc  ActiveDisplayYMinimum=-59.27589767770079  ActiveDisplayYMaximum=564.40900084144926
  wires:
  [diode_JH_temp_invQ1] -> Bus Creator6/1  "diode_JH_temp_invQ1"
  [diode_ploss_invQ1] -> diode power losses INV Q1/1  "diode_ploss_invQ1"
  Bus Creator2/1 -> igbt power losses INV Q1/4
  [diode_HA_temp_invQ1] -> Bus Creator6/2  "diode_HA_temp_invQ1"
  [igbt_current_invQ1] -> igbt power losses INV Q1/2  "igbt_current_invQ1"
  [igbt_HA_temp_invQ1] -> Bus Creator2/2  "igbt_HA_temp_invQ1"
  Bus Creator1/1 -> igbt power losses INV Q2/4
  [igbt_voltage_invQ1] -> igbt power losses INV Q1/3  "igbt_voltage_invQ1"
  [igbt_JH_temp_invQ2] -> Bus Creator1/1  "igbt_JH_temp_invQ2"
  [igbt_current_invQ2] -> igbt power losses INV Q2/2  "igbt_current_invQ2"
  [igbt_ploss_invQ1] -> igbt power losses INV Q1/1  "igbt_ploss_invQ1"
  [igbt_HA_temp_invQ2] -> Bus Creator1/2  "igbt_HA_temp_invQ2"
  [igbt_JH_temp_invQ1] -> Bus Creator2/1  "igbt_JH_temp_invQ1"
  [igbt_ploss_invQ2] -> igbt power losses INV Q2/1  "igbt_ploss_invQ2"
  [igbt_voltage_invQ2] -> igbt power losses INV Q2/3  "igbt_voltage_invQ2"
  Bus Creator6/1 -> diode power losses INV Q1/2

== system mpc_psm/scopes/scopes_for_mosfet_based_inverter ==
  Bus Creator8 : BusCreator  Inputs=2
  Bus Creator9 : BusCreator  Inputs=2
  mosfet power losses INV Q1 : Scope  NumInputPorts=4
      settings: SampleTime=tc  ActiveDisplayYMinimum=-32.258190719935513  ActiveDisplayYMaximum=388.05311151106906  DataLoggingVariableName=ScopeData28
  mosfet power losses INV Q2 : Scope  NumInputPorts=4
      settings: SampleTime=tc  ActiveDisplayYMinimum=-60.051099059926763  ActiveDisplayYMaximum=540.45256909803  DataLoggingVariableName=ScopeData29
  wires:
  [mosfet_JH_temp_invQ1] -> Bus Creator8/1  "mosfet_JH_temp_invQ1"
  Bus Creator9/1 -> mosfet power losses INV Q2/4
  [mosfet_HA_temp_invQ2] -> Bus Creator9/2  "mosfet_HA_temp_invQ2"
  [mosfet_HA_temp_invQ1] -> Bus Creator8/2  "mosfet_HA_temp_invQ1"
  [mosfet_ploss_invQ2] -> mosfet power losses INV Q2/1  "mosfet_ploss_invQ2"
  [mosfet_JH_temp_invQ2] -> Bus Creator9/1  "mosfet_JH_temp_invQ2"
  [mosfet_current_invQ2] -> mosfet power losses INV Q2/3  "mosfet_current_invQ2"
  [mosfet_ploss_invQ1] -> mosfet power losses INV Q1/1  "mosfet_ploss_invQ1"
  [mosfet_voltage_invQ2] -> mosfet power losses INV Q2/2  "mosfet_voltage_invQ2"
  [mosfet_current_invQ1] -> mosfet power losses INV Q1/3  "mosfet_current_invQ1"
  Bus Creator8/1 -> mosfet power losses INV Q1/4
  [mosfet_voltage_invQ1] -> mosfet power losses INV Q1/2  "mosfet_voltage_invQ1"

== system mpc_psm/inv_psm_mod1/inverter/inverter ==
  gate_cmds_uvw : Inport
  PS Terminator : fl_lib/Physical Signals/Sinks/PS Terminator
  PS Terminator1 : fl_lib/Physical Signals/Sinks/PS Terminator
  Simulink-PS Converter : nesl_utility/Simulink-PS Converter  PhysicalDomain=network_engine_domain  SubClassName=ps_input  LeftPortType=input  RightPortType=output  PseudoPeriodic=off  Frequencies=[]  NoiseDistribution=none  NoiseParameters=[]  Unit=V  AffineConversion=off  FilteringAndDerivatives=provide  SimscapeFilterOrder=1  InputFilterTimeConstant=0.001  UdotUserProvided=0
  Three-Phase Bridge (ideal) : ideal_bridges_lib/Three-Phase Bridge (ideal)  Vth=2.5 V  Ron=1e-3 Ohm  Goff=1e-6 1/Ohm  cap_dc=ideal_bridges.onoff.off  Cdc=2e-3 F  Vdc0=0 V  ind_ac=ideal_bridges.onoff.off  L=1e-3 H  RL=10e-3 Ohm  vdc_specify=off  vdc_priority=None  vdc=0 V  vdc_nominal_specify=off  vdc_nominal_value=1  vdc_nominal_unit=V  ic_specify=off  ic_priority=None  ic=0 A  ic_nominal_specify=off  ic_nominal_value=1  ic_nominal_unit=A  vm_a_specify=off  vm_a_priority=None  vm_a=0 V  vm_a_nominal_specify=off  vm_a_nominal_value=1  vm_a_nominal_unit=V  vm_b_specify=off  vm_b_priority=None  vm_b=0 V  vm_b_nominal_specify=off  vm_b_nominal_value=1  vm_b_nominal_unit=V  vm_c_specify=off  vm_c_priority=None  vm_c=0 V  vm_c_nominal_specify=off  vm_c_nominal_value=1  vm_c_nominal_unit=V  i_ah_specify=off  i_ah_priority=None  i_ah=0 A  i_ah_nominal_specify=off  i_ah_nominal_value=1  i_ah_nominal_unit=A  i_al_specify=off  i_al_priority=None  i_al=0 A  i_al_nominal_specify=off  i_al_nominal_value=1  i_al_nominal_unit=A  i_bh_specify=off  i_bh_priority=None  i_bh=0 A  i_bh_nominal_specify=off  i_bh_nominal_value=1  i_bh_nominal_unit=A  i_bl_specify=off  i_bl_priority=None  i_bl=0 A  i_bl_nominal_specify=off  i_bl_nominal_value=1  i_bl_nominal_unit=A  i_ch_specify=off  i_ch_priority=None  i_ch=0 A  i_ch_nominal_specify=off  i_ch_nominal_value=1  i_ch_nominal_unit=A  i_cl_specify=off  i_cl_priority=None  i_cl=0 A  i_cl_nominal_specify=off  i_cl_nominal_value=1  i_cl_nominal_unit=A  i_a_specify=off  i_a_priority=None  i_a=0 A  i_a_nominal_specify=off  i_a_nominal_value=1  i_a_nominal_unit=A  i_b_specify=off  i_b_priority=None  i_b=0 A  i_b_nominal_specify=off  i_b_nominal_value=1  i_b_nominal_unit=A  i_c_specify=off  i_c_priority=None  i_c=0 A  i_c_nominal_specify=off  i_c_nominal_value=1  i_c_nominal_unit=A
  dead_time_generator_cmos_simulink : dead_time_generator_cmos_simulink/dead_time_generator_cmos_simulink  ts=param.glb_time.tc  positive_voltage_rail=15  dead_time=param.glb_time.dead_time_INV
  timer : Subsystem  mask{f=param.glb_time.fPWM_INV, m_up=0.98, m_low=0.02, dead_time=param.glb_time.dead_time_INV, pos_cmd_gate=15, neg_cmd_gate=-10, polarity=1, tc=param.glb_time.tc, double_sampling=param.glb_time.TRGO_INV_double_update}
      mask prompts: f "Frequency (Hz)"; m_up "Max Input Modulation Value"; m_low "Min Input Modulation Value"; dead_time "Dead Time (s)"; pos_cmd_gate "Positive Gate Voltage (V)"; neg_cmd_gate "Negative Gate Voltage (V)"; polarity "Polarity (pu)"; tc "Sampling time"
  u : PMIOPort  Side=Left
  v : PMIOPort  Port=2  Side=Left
  w : PMIOPort  Port=3  Side=Left
  udc(+) : PMIOPort  Port=4  Side=Right
  udc(-) : PMIOPort  Port=5  Side=Right
  tag scope: TRGO_inv_module_1=global
  wires:
  dead_time_generator_cmos_simulink/1 -> Simulink-PS Converter/1
  timer/1(TRGO) -> [TRGO_inv_module_1]
  [time_inv_module_1] -> timer/1(time_source)
  gate_cmds_uvw/1 -> dead_time_generator_cmos_simulink/1
  connections:
  udc(+)/RConn1 -- Three-Phase Bridge (ideal)/LConn1
  udc(-)/RConn1 -- Three-Phase Bridge (ideal)/LConn2
  u/RConn1 -- Three-Phase Bridge (ideal)/RConn1
  v/RConn1 -- Three-Phase Bridge (ideal)/RConn2
  w/RConn1 -- Three-Phase Bridge (ideal)/RConn3
  PS Terminator/LConn1 -- Three-Phase Bridge (ideal)/LConn3
  PS Terminator1/LConn1 -- Three-Phase Bridge (ideal)/LConn4
  Simulink-PS Converter/RConn1 -- Three-Phase Bridge (ideal)/RConn4

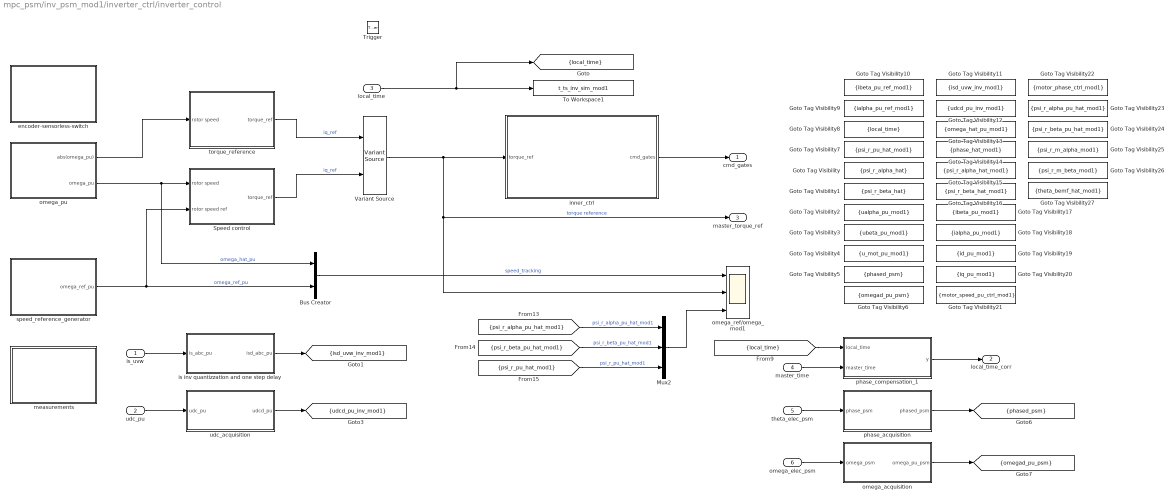
== system mpc_psm/inv_psm_mod1/inverter_ctrl/inverter_control ==
  is_uvw : Inport
  udc_pu : Inport  Port=2
  local_time : Inport  Port=3
  master_time : Inport  Port=4
  theta_elec_psm : Inport  Port=5
  omega_elec_psm : Inport  Port=6
  Trigger : TriggerPort  VariantControl=(inherit)  PortDimensions=1
  Bus Creator : BusCreator  Inputs=2
  Goto Tag Visibility : GotoTagVisibility  GotoTag=psi_r_alpha_hat
  Goto Tag Visibility1 : GotoTagVisibility  GotoTag=psi_r_beta_hat
  Goto Tag Visibility10 : GotoTagVisibility  GotoTag=ibeta_pu_ref_mod1
  Goto Tag Visibility11 : GotoTagVisibility  GotoTag=isd_uvw_inv_mod1
  Goto Tag Visibility12 : GotoTagVisibility  GotoTag=udcd_pu_inv_mod1
  Goto Tag Visibility13 : GotoTagVisibility  GotoTag=omega_hat_pu_mod1
  Goto Tag Visibility14 : GotoTagVisibility  GotoTag=phase_hat_mod1
  Goto Tag Visibility15 : GotoTagVisibility  GotoTag=psi_r_alpha_hat_mod1
  Goto Tag Visibility16 : GotoTagVisibility  GotoTag=psi_r_beta_hat_mod1
  Goto Tag Visibility17 : GotoTagVisibility  GotoTag=ibeta_pu_mod1
  Goto Tag Visibility18 : GotoTagVisibility  GotoTag=ialpha_pu_mod1
  Goto Tag Visibility19 : GotoTagVisibility  GotoTag=id_pu_mod1
  Goto Tag Visibility2 : GotoTagVisibility  GotoTag=ualpha_pu_mod1
  Goto Tag Visibility20 : GotoTagVisibility  GotoTag=iq_pu_mod1
  Goto Tag Visibility21 : GotoTagVisibility  GotoTag=motor_speed_pu_ctrl_mod1
  Goto Tag Visibility22 : GotoTagVisibility  GotoTag=motor_phase_ctrl_mod1
  Goto Tag Visibility23 : GotoTagVisibility  GotoTag=psi_r_alpha_pu_hat_mod1
  Goto Tag Visibility24 : GotoTagVisibility  GotoTag=psi_r_beta_pu_hat_mod1
  Goto Tag Visibility25 : GotoTagVisibility  GotoTag=psi_r_m_alpha_mod1
  Goto Tag Visibility26 : GotoTagVisibility  GotoTag=psi_r_m_beta_mod1
  Goto Tag Visibility27 : GotoTagVisibility  GotoTag=theta_bemf_hat_mod1
  Goto Tag Visibility3 : GotoTagVisibility  GotoTag=ubeta_pu_mod1
  Goto Tag Visibility4 : GotoTagVisibility  GotoTag=u_mot_pu_mod1
  Goto Tag Visibility5 : GotoTagVisibility  GotoTag=phased_psm
  Goto Tag Visibility6 : GotoTagVisibility  GotoTag=omegad_pu_psm
  Goto Tag Visibility7 : GotoTagVisibility  GotoTag=psi_r_pu_hat_mod1
  Goto Tag Visibility8 : GotoTagVisibility  GotoTag=local_time
  Goto Tag Visibility9 : GotoTagVisibility  GotoTag=ialpha_pu_ref_mod1
  Mux2 : Mux  Inputs=3
  Speed control : Subsystem
  To Workspace1 : ToWorkspace  VariableName=t_ts_inv_sim_mod1  SampleTime=-1
      settings: MaxDataPoints=param.glb_time.Ns_inv
  Variant Source : VariantSource  VariantControls={param.psm.mode.use_torque_curve == 1, param.psm.mode.use_speed_control == 1}
  encoder-sensorless-switch : Subsystem
  inner_ctrl : Subsystem
  is inv quantizzation and one step delay : Subsystem
  measurements : Subsystem
  omega_acquisition : Subsystem
  omega_pu : Subsystem
  omega_ref/omega_mod1 : Scope  NumInputPorts=3
      settings: ActiveDisplayYMinimum=-1.7949249844307968  ActiveDisplayYMaximum=1.3113178143582995  DataLoggingVariableName=ScopeData3
  phase_acquisition : Subsystem
  phase_compensation_1 : Subsystem
  speed_reference_generator : Subsystem
  torque_reference : Subsystem
  udc_acquisition : Subsystem
  cmd_gates : Outport  VectorParamsAs1DForOutWhenUnconnected=off
  local_time_corr : Outport  Port=2
  master_torque_ref : Outport  Port=3  VectorParamsAs1DForOutWhenUnconnected=off
  tag scope: isd_uvw_inv_mod1=scoped, local_time=scoped, omegad_pu_psm=scoped, phased_psm=scoped, udcd_pu_inv_mod1=scoped
  wires:
  speed_reference_generator/1(omega_ref_pu) -> Speed control/2(rotor speed ref), Bus Creator/2  "omega_ref_pu"
  Bus Creator/1 -> omega_ref/omega_mod1/1  "speed_tracking"
  Variant Source/1 -> master_torque_ref/1, omega_ref/omega_mod1/2, inner_ctrl/1(torque_ref)  "torque reference"
  [psi_r_alpha_pu_hat_mod1] -> Mux2/1  "psi_r_alpha_pu_hat_mod1"
  [psi_r_beta_pu_hat_mod1] -> Mux2/2  "psi_r_beta_pu_hat_mod1"
  Mux2/1 -> omega_ref/omega_mod1/3
  [psi_r_pu_hat_mod1] -> Mux2/3  "psi_r_pu_hat_mod1"
  omega_pu/2(omega_pu) -> Bus Creator/1, Speed control/1(rotor speed)  "omega_hat_pu"
  omega_pu/1(abs(omega_pu)) -> torque_reference/1(rotor speed)
  torque_reference/1(torque_ref) -> Variant Source/1  "iq_ref"
  Speed control/1(torque_ref) -> Variant Source/2  "iq_ref"
  udc_acquisition/1(udcd_pu) -> [udcd_pu_inv_mod1]
  udc_pu/1 -> udc_acquisition/1(udc_pu)
  is_uvw/1 -> is inv quantizzation and one step delay/1(is_abc_pu)
  is inv quantizzation and one step delay/1(isd_abc_pu) -> [isd_uvw_inv_mod1]
  local_time/1 -> To Workspace1/1, [local_time]
  inner_ctrl/1(cmd_gates) -> cmd_gates/1
  master_time/1 -> phase_compensation_1/2(master_time)
  [local_time] -> phase_compensation_1/1(local_time)
  phase_compensation_1/1(y) -> local_time_corr/1
  theta_elec_psm/1 -> phase_acquisition/1(phase_psm)
  omega_elec_psm/1 -> omega_acquisition/1(omega_psm)
  phase_acquisition/1(phased_psm) -> [phased_psm]
  omega_acquisition/1(omega_pu_psm) -> [omegad_pu_psm]
